simulink model "fsd_suspension"  (R2024b)
settings: Solver=ode15s  StartTime=0.0  StopTime=Tsim  FixedStep=Ts  MaxStep=1e-4  RelTol=1e-4
values from neighbouring files (symbols this model uses):
  b1 = 3500    [FSD_Analysis.m]    (also in FSD_Parameter_Sweep.m)
  b2 = 100    [FSD_Analysis.m]    (also in FSD_Parameter_Sweep.m)
  C_base = 1500    [FSD_Analysis.m]
  C_fsd = 2000    [FSD_Analysis.m]
  K_fsd = 50000    [FSD_Analysis.m]
  tau = 1/(2*pi*fc)    (= 0.0530516476973)    [FSD_Analysis.m]
undefined symbols (not defined in the file or in its folder): c_high, c_low
libraries: fl_lib x27, nesl_utility x21, sdl_lib x3
settings Model: Creator=Dinulkar  LastModifiedBy=dinul
settings DataIOCC: ReturnWorkspaceOutputs=off

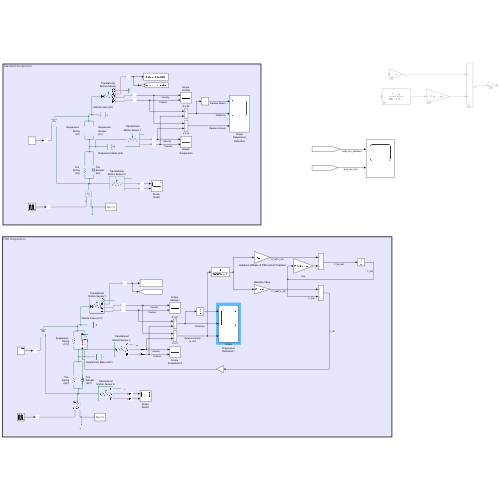
[thumbnail: Simulink's stored preview of the top-level diagram]
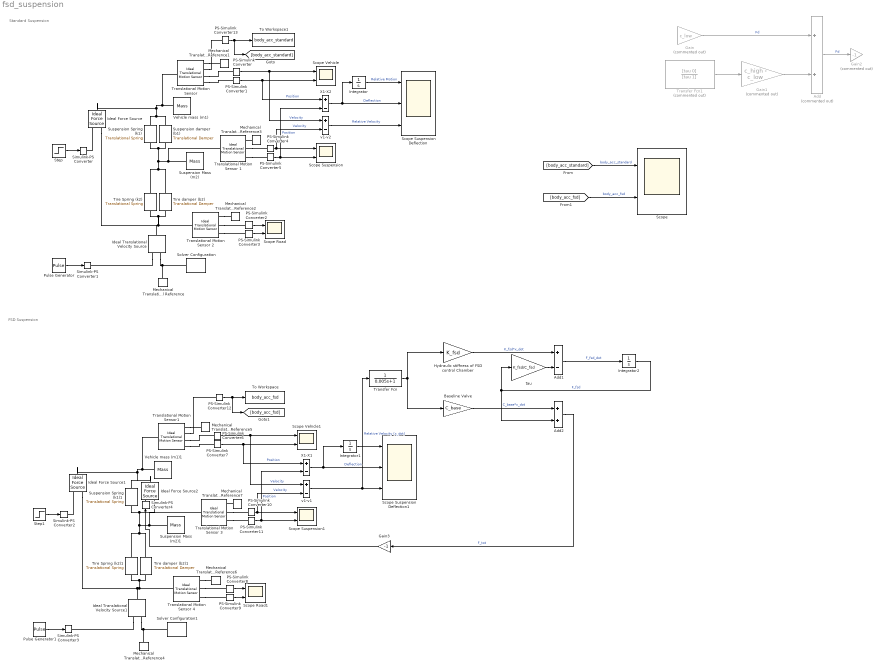
== system fsd_suspension ==
  note: FSD Suspension
  note: Standard Suspension
  Add : Sum  Commented=on
  Add1 : Sum  Inputs=+-
  Add2 : Sum
  Baseline Valve : Gain  Gain=C_base
  Gain : Gain  Commented=on  Gain=c_low
  Gain1 : Gain  Commented=on  Gain=c_high - c_low
  Gain2 : Gain  Commented=on  Gain=-1
  Gain3 : Gain  Gain=-1
  Hydraulic stiffness of FSD control Chamber : Gain  Gain=K_fsd
  Ideal Force Source : fl_lib/Mechanical/Mechanical Sources/Ideal Force Source
  Ideal Force Source1 : fl_lib/Mechanical/Mechanical Sources/Ideal Force Source
  Ideal Force Source2 : fl_lib/Mechanical/Mechanical Sources/Ideal Force Source
  Ideal Translational Velocity Source : fl_lib/Mechanical/Mechanical Sources/Ideal Translational Velocity Source
  Ideal Translational Velocity Source1 : fl_lib/Mechanical/Mechanical Sources/Ideal Translational Velocity Source
  Integrator : Integrator
  Integrator1 : Integrator
  Integrator2 : Integrator
  Mechanical Translational Reference{,1..7} (8 alike) : fl_lib/Mechanical/Translational Elements/Mechanical Translational Reference
  PS-Simulink Converter{,1..11} (12 alike) : nesl_utility/PS-Simulink Converter  PhysicalDomain=network_engine_domain  SubClassName=ps_output  LeftPortType=input  RightPortType=output  PseudoPeriodic=off  Frequencies=[]  VectorFormat=inherit  Unit=inherit  AffineConversion=off
  PS-Simulink Converter12 : nesl_utility/PS-Simulink Converter  PhysicalDomain=network_engine_domain  SubClassName=ps_output  LeftPortType=input  RightPortType=output  PseudoPeriodic=off  Frequencies=[]  VectorFormat=1-D array  Unit=inherit  AffineConversion=off
  PS-Simulink Converter13 : nesl_utility/PS-Simulink Converter  PhysicalDomain=network_engine_domain  SubClassName=ps_output  LeftPortType=input  RightPortType=output  PseudoPeriodic=off  Frequencies=[]  VectorFormat=1-D array  Unit=inherit  AffineConversion=off
  Pulse Generator : DiscretePulseGenerator  PulseType=Time based  Amplitude=0.05  PulseWidth=10  PhaseDelay=1  SampleTime=0.001
  Pulse Generator1 : DiscretePulseGenerator  PulseType=Time based  Amplitude=0.05  PulseWidth=10  PhaseDelay=1  SampleTime=0.001
  Scope : Scope  NumInputPorts=2
  Scope Suspension Deflection : Scope  NumInputPorts=3
  Scope Suspension Deflection1 : Scope  NumInputPorts=3
  Scope Road : Scope  NumInputPorts=2
  Scope Road1 : Scope  NumInputPorts=2
  Scope Suspension : Scope  NumInputPorts=2
  Scope Suspension1 : Scope  NumInputPorts=2
  Scope Vehicle : Scope  NumInputPorts=2
  Scope Vehicle1 : Scope  NumInputPorts=2
  Simulink-PS Converter : nesl_utility/Simulink-PS Converter  PhysicalDomain=network_engine_domain  SubClassName=ps_input  LeftPortType=input  RightPortType=output  PseudoPeriodic=off  Frequencies=[]  NoiseDistribution=none  NoiseParameters=[]  Unit=N  AffineConversion=on  FilteringAndDerivatives=zero  SimscapeFilterOrder=1  InputFilterTimeConstant=0.001  UdotUserProvided=0
  Simulink-PS Converter1 : nesl_utility/Simulink-PS Converter  PhysicalDomain=network_engine_domain  SubClassName=ps_input  LeftPortType=input  RightPortType=output  PseudoPeriodic=off  Frequencies=[]  NoiseDistribution=none  NoiseParameters=[]  Unit=m/s  AffineConversion=on  FilteringAndDerivatives=zero  SimscapeFilterOrder=1  InputFilterTimeConstant=0.001  UdotUserProvided=0
  Simulink-PS Converter2 : nesl_utility/Simulink-PS Converter  PhysicalDomain=network_engine_domain  SubClassName=ps_input  LeftPortType=input  RightPortType=output  PseudoPeriodic=off  Frequencies=[]  NoiseDistribution=none  NoiseParameters=[]  Unit=N  AffineConversion=on  FilteringAndDerivatives=filter  SimscapeFilterOrder=1  InputFilterTimeConstant=0.01  UdotUserProvided=0
  Simulink-PS Converter3 : nesl_utility/Simulink-PS Converter  PhysicalDomain=network_engine_domain  SubClassName=ps_input  LeftPortType=input  RightPortType=output  PseudoPeriodic=off  Frequencies=[]  NoiseDistribution=none  NoiseParameters=[]  Unit=m/s  AffineConversion=on  FilteringAndDerivatives=filter  SimscapeFilterOrder=1  InputFilterTimeConstant=0.01  UdotUserProvided=0
  Simulink-PS Converter4 : nesl_utility/Simulink-PS Converter  PhysicalDomain=network_engine_domain  SubClassName=ps_input  LeftPortType=input  RightPortType=output  PseudoPeriodic=off  Frequencies=[]  NoiseDistribution=none  NoiseParameters=[]  Unit=N  AffineConversion=off  FilteringAndDerivatives=zero  SimscapeFilterOrder=1  InputFilterTimeConstant=0.001  UdotUserProvided=0
  Solver Configuration : nesl_utility/Solver Configuration  PhysicalDomain=network_engine_domain  SubClassName=solver  LeftPortType=input  RightPortType=generic  Tones=[]  Harmonics=[]  SimulateNoise=off  Profile=off  UseLocalSampling=off  EnableSwitchedLinearOptims=on  FrequencyDomain=off  UseCCode=off  RelTol=0.001  AbsTol=0.001  MinStep=1e-09  ToWorkspace=off  RevertToSquareIcSolve=off  NumHomotopyIterations=100  PhasorMode=off  PhasorModeNumHarmonics=1  ConsistencySolver=NEWTON_XTOL_AFTER_FTOL  IndexReductionMethod=DerivativeReplacement  DoDC=off  ResidualTolerance=1e-09  ConsistencyTolSource=GLOBAL  ConsistencyAbsTol=0.001  ConsistencyRelTol=0.001  ConsistencyTolFactor=0.001  UseLocalSolver=off  LocalSolverChoice=NE_BACKWARD_EULER_ADVANCER  ResolveIndetEquations=on  FunctionEvalNumThread=1  LocalSolverSampleTime=0.001  DoFixedCost=off  MaxNonlinIter=3  MaxModeIter=2  ComputeImpulses=off  ImpulseIterations=2  LinearAlgebra=auto  LinearAlgebraNumThread=0  EquationFormulation=NE_TIME_EF  DelaysMemoryBudget=1024  AutomaticFiltering=on  FilteringTimeConstant=0.001  PartitionStorageMethod=AS_NEEDED  PartitionMemoryBudget=1024  PartitionMethod=ROBUST  MultibodyUseLocalSolver=off  MultibodyLocalSolverChoice=ODE1  MultibodyLocalSolverSampleTime=0.001
  Solver Configuration1 : nesl_utility/Solver Configuration  PhysicalDomain=network_engine_domain  SubClassName=solver  LeftPortType=input  RightPortType=generic  Tones=[]  Harmonics=[]  SimulateNoise=off  Profile=off  UseLocalSampling=off  EnableSwitchedLinearOptims=on  FrequencyDomain=off  UseCCode=off  RelTol=0.001  AbsTol=0.001  MinStep=1e-09  ToWorkspace=off  RevertToSquareIcSolve=off  NumHomotopyIterations=100  PhasorMode=off  PhasorModeNumHarmonics=1  ConsistencySolver=NEWTON_XTOL_AFTER_FTOL  IndexReductionMethod=DerivativeReplacement  DoDC=off  ResidualTolerance=1e-09  ConsistencyTolSource=GLOBAL  ConsistencyAbsTol=0.001  ConsistencyRelTol=0.001  ConsistencyTolFactor=0.001  UseLocalSolver=off  LocalSolverChoice=NE_BACKWARD_EULER_ADVANCER  ResolveIndetEquations=on  FunctionEvalNumThread=1  LocalSolverSampleTime=0.001  DoFixedCost=off  MaxNonlinIter=3  MaxModeIter=2  ComputeImpulses=off  ImpulseIterations=2  LinearAlgebra=auto  LinearAlgebraNumThread=0  EquationFormulation=NE_TIME_EF  DelaysMemoryBudget=1024  AutomaticFiltering=on  FilteringTimeConstant=0.001  PartitionStorageMethod=AS_NEEDED  PartitionMemoryBudget=1024  PartitionMethod=ROBUST  MultibodyUseLocalSolver=off  MultibodyLocalSolverChoice=ODE1  MultibodyLocalSolverSampleTime=0.001
  Step : Step  After=100  SampleTime=0
  Step1 : Step  After=100  SampleTime=0
  Suspension Spring (k1) : fl_lib/Mechanical/Translational Elements/Translational Spring  spr_rate=k1 N/m  v_specify=off  v_priority=None  v=0 m/s  v_nominal_specify=off  v_nominal_value=1  v_nominal_unit=m/s  f_specify=off  f_priority=None  f=0 N  f_nominal_specify=off  f_nominal_value=1  f_nominal_unit=N  x_specify=off  x_priority=High  x=0 m  x_nominal_specify=off  x_nominal_value=1  x_nominal_unit=m
  Suspension Spring (k1)1 : fl_lib/Mechanical/Translational Elements/Translational Spring  spr_rate=k1 N/m  v_specify=off  v_priority=None  v=0 m/s  v_nominal_specify=off  v_nominal_value=1  v_nominal_unit=m/s  f_specify=off  f_priority=None  f=0 N  f_nominal_specify=off  f_nominal_value=1  f_nominal_unit=N  x_specify=off  x_priority=High  x=0 m  x_nominal_specify=off  x_nominal_value=1  x_nominal_unit=m
  Suspension damper (b1) : sdl_lib/Couplings & Drives/Springs & Dampers/Translational Damper  D=b1 N*s/m  thermal_port=simscape.enum.thermaleffects.omit  thermal_mass=50 kJ/K  temperature_specify=off  temperature_priority=High  temperature=300 K  temperature_nominal_specify=off  temperature_nominal_value=1  temperature_nominal_unit=K
  Suspension Mass (m2) : fl_lib/Mechanical/Translational Elements/Mass  mass=m2 kg  num_ports=foundation.enum.numPorts2.one  v_specify=off  v_priority=High  v=0 m/s  v_nominal_specify=off  v_nominal_value=1  v_nominal_unit=m/s  f_specify=off  f_priority=None  f=0 N  f_nominal_specify=off  f_nominal_value=1  f_nominal_unit=N
  Suspension Mass (m2)1 : fl_lib/Mechanical/Translational Elements/Mass  mass=m2 kg  num_ports=foundation.enum.numPorts2.one  v_specify=off  v_priority=High  v=0 m/s  v_nominal_specify=off  v_nominal_value=1  v_nominal_unit=m/s  f_specify=off  f_priority=None  f=0 N  f_nominal_specify=off  f_nominal_value=1  f_nominal_unit=N
  Tire Spring (k2) : fl_lib/Mechanical/Translational Elements/Translational Spring  spr_rate=k2 N/m  v_specify=off  v_priority=None  v=0 m/s  v_nominal_specify=off  v_nominal_value=1  v_nominal_unit=m/s  f_specify=off  f_priority=None  f=0 N  f_nominal_specify=off  f_nominal_value=1  f_nominal_unit=N  x_specify=off  x_priority=High  x=0 m  x_nominal_specify=off  x_nominal_value=1  x_nominal_unit=m
  Tire Spring (k2)1 : fl_lib/Mechanical/Translational Elements/Translational Spring  spr_rate=k2 N/m  v_specify=off  v_priority=None  v=0 m/s  v_nominal_specify=off  v_nominal_value=1  v_nominal_unit=m/s  f_specify=off  f_priority=None  f=0 N  f_nominal_specify=off  f_nominal_value=1  f_nominal_unit=N  x_specify=off  x_priority=High  x=0 m  x_nominal_specify=off  x_nominal_value=1  x_nominal_unit=m
  Tire damper (b2) : sdl_lib/Couplings & Drives/Springs & Dampers/Translational Damper  D=b2 N*s/m  thermal_port=simscape.enum.thermaleffects.omit  thermal_mass=50 kJ/K  temperature_specify=off  temperature_priority=High  temperature=300 K  temperature_nominal_specify=off  temperature_nominal_value=1  temperature_nominal_unit=K
  Tire damper (b2)1 : sdl_lib/Couplings & Drives/Springs & Dampers/Translational Damper  D=b2 N*s/m  thermal_port=simscape.enum.thermaleffects.omit  thermal_mass=50 kJ/K  temperature_specify=off  temperature_priority=High  temperature=300 K  temperature_nominal_specify=off  temperature_nominal_value=1  temperature_nominal_unit=K
  To Workspace : ToWorkspace  VariableName=body_acc_fsd  SaveFormat=Structure With Time  SampleTime=-1
  To Workspace1 : ToWorkspace  VariableName=body_acc_standard  SaveFormat=Structure With Time  SampleTime=-1
  Transfer Fcn : TransferFcn  Denominator=[0.005 1]
  Transfer Fcn1 : TransferFcn  Commented=on  Numerator=[tau 0]  Denominator=[tau 1]
  Translational Motion Sensor : fl_lib/Mechanical/Mechanical Sensors/Ideal Translational Motion Sensor  reference=foundation.enum.MeasurementReference.difference  acceleration_port=true  velocity_port=true  position_port=true  offset=0 m
      settings: InternalSimscapePortConfiguration="{\"Bottom\":[],\"Left\":[{\"id\":\"R\",\"label\":\"R\",\"type\":\"foundation.mechanical.translational.translational\"}],\"Right\":[{\"id\":\"C\",\"label\":\"C\",\"type\":\"foundation.mechanical.translational.translational\"},{\"id\":\"A\",\"label\":\"A\",\"type\":\"output\"},{\"id\":\"V\",\"label\":\"V\",\"type\":\"output\"},{\"id\":\"P\",\"label\":\"P\",\"type\":\"output\"}],\"Top\":[]}"
  Translational Motion Sensor {1..4} (4 alike) : fl_lib/Mechanical/Mechanical Sensors/Ideal Translational Motion Sensor  reference=foundation.enum.MeasurementReference.difference  acceleration_port=false  velocity_port=true  position_port=true  offset=0 m
  Translational Motion Sensor1 : fl_lib/Mechanical/Mechanical Sensors/Ideal Translational Motion Sensor  reference=foundation.enum.MeasurementReference.difference  acceleration_port=true  velocity_port=true  position_port=true  offset=0 m
      settings: InternalSimscapePortConfiguration="{\"Bottom\":[],\"Left\":[{\"id\":\"R\",\"label\":\"R\",\"type\":\"foundation.mechanical.translational.translational\"}],\"Right\":[{\"id\":\"C\",\"label\":\"C\",\"type\":\"foundation.mechanical.translational.translational\"},{\"id\":\"A\",\"label\":\"A\",\"type\":\"output\"},{\"id\":\"V\",\"label\":\"V\",\"type\":\"output\"},{\"id\":\"P\",\"label\":\"P\",\"type\":\"output\"}],\"Top\":[]}"
  Vehicle mass (m1) : fl_lib/Mechanical/Translational Elements/Mass  mass=m1 kg  num_ports=foundation.enum.numPorts2.one  v_specify=off  v_priority=High  v=0 m/s  v_nominal_specify=off  v_nominal_value=1  v_nominal_unit=m/s  f_specify=off  f_priority=None  f=0 N  f_nominal_specify=off  f_nominal_value=1  f_nominal_unit=N
  Vehicle mass (m1)1 : fl_lib/Mechanical/Translational Elements/Mass  mass=m1 kg  num_ports=foundation.enum.numPorts2.one  v_specify=off  v_priority=High  v=0 m/s  v_nominal_specify=off  v_nominal_value=1  v_nominal_unit=m/s  f_specify=off  f_priority=None  f=0 N  f_nominal_specify=off  f_nominal_value=1  f_nominal_unit=N
  X1-X1 : Sum  Inputs=+-
  X1-X2 : Sum  Inputs=+-
  tau : Gain  Gain=K_fsd/C_fsd
  v1-v1 : Sum  Inputs=+-
  v1-v2 : Sum  Inputs=+-
  wires:
  Step/1 -> Simulink-PS Converter/1
  Pulse Generator/1 -> Simulink-PS Converter1/1
  PS-Simulink Converter/1 -> v1-v2/1, Scope Vehicle/1  "Velocity"
  PS-Simulink Converter1/1 -> X1-X2/1, Scope Vehicle/2  "Position"
  PS-Simulink Converter2/1 -> Scope Road/1
  PS-Simulink Converter3/1 -> Scope Road/2
  PS-Simulink Converter5/1 -> X1-X2/2, Scope Suspension/2  "Position"
  PS-Simulink Converter4/1 -> v1-v2/2, Scope Suspension/1  "Velocity"
  X1-X2/1 -> Scope Suspension Deflection/2, Integrator/1  "Deflection"
  v1-v1/1 -> Transfer Fcn/1, Scope Suspension Deflection1/3  "Relative Velocity (x_dot)"
  Integrator/1 -> Scope Suspension Deflection/1  "Relative Motion"
  Integrator1/1 -> Scope Suspension Deflection1/1
  X1-X1/1 -> Integrator1/1, Scope Suspension Deflection1/2  "Deflection"
  PS-Simulink Converter10/1 -> Scope Suspension1/1, v1-v1/2  "Velocity"
  PS-Simulink Converter11/1 -> Scope Suspension1/2, X1-X1/2  "Position"
  PS-Simulink Converter9/1 -> Scope Road1/2
  PS-Simulink Converter8/1 -> Scope Road1/1
  PS-Simulink Converter7/1 -> Scope Vehicle1/2, X1-X1/1  "Position"
  PS-Simulink Converter6/1 -> Scope Vehicle1/1, v1-v1/1  "Velocity"
  Pulse Generator1/1 -> Simulink-PS Converter3/1
  Step1/1 -> Simulink-PS Converter2/1
  PS-Simulink Converter12/1 -> [body_acc_fsd], To Workspace/1
  PS-Simulink Converter13/1 -> [body_acc_standard], To Workspace1/1
  v1-v2/1 -> Scope Suspension Deflection/3  "Relative Velocity"
  [body_acc_standard] -> Scope/1  "body_acc_standard"
  [body_acc_fsd] -> Scope/2  "body_acc_fsd"
  Hydraulic stiffness of FSD control Chamber/1 -> Add1/1  "K_fsd*x_dot"
  Add1/1 -> Integrator2/1  "F_fsd_dot"
  Integrator2/1 -> Add2/2, tau/1  "F_fsd"
  tau/1 -> Add1/2
  Add2/1 -> Gain3/1  "F_tot"
  Gain1/1 -> Add/2
  Gain/1 -> Add/1  "Fd"
  Add/1 -> Gain2/1  "Fd"
  Transfer Fcn1/1 -> Gain1/1
  Transfer Fcn/1 -> Baseline Valve/1, Hydraulic stiffness of FSD control Chamber/1
  Baseline Valve/1 -> Add2/1  "C_base*x_dot"
  Gain3/1 -> Simulink-PS Converter4/1
  connections:
  Simulink-PS Converter/RConn1 -- Ideal Force Source/RConn1
  Suspension Spring (k1)/LConn1 -- Ideal Force Source/LConn1 -- Translational Motion Sensor/LConn1 -- Vehicle mass (m1)/LConn1 -- Suspension damper (b1)/LConn1
  Suspension Spring (k1)/RConn1 -- Tire damper (b2)/LConn1 -- Tire Spring (k2)/LConn1 -- Translational Motion Sensor 1/LConn1 -- Suspension Mass (m2)/LConn1 -- Suspension damper (b1)/RConn1
  Ideal Translational Velocity Source/RConn1 -- Simulink-PS Converter1/RConn1
  Tire Spring (k2)/RConn1 -- Ideal Force Source/RConn2 -- Ideal Translational Velocity Source/LConn1 -- Translational Motion Sensor 2/LConn1 -- Tire damper (b2)/RConn1
  Mechanical Translational Reference/LConn1 -- Ideal Translational Velocity Source/RConn2 -- Solver Configuration/RConn1
  Translational Motion Sensor/RConn1 -- Mechanical Translational Reference1/LConn1
  Translational Motion Sensor 2/RConn1 -- Mechanical Translational Reference2/LConn1
  Translational Motion Sensor/RConn3 -- PS-Simulink Converter/LConn1
  Translational Motion Sensor/RConn4 -- PS-Simulink Converter1/LConn1
  Translational Motion Sensor 2/RConn2 -- PS-Simulink Converter2/LConn1
  Translational Motion Sensor 2/RConn3 -- PS-Simulink Converter3/LConn1
  Translational Motion Sensor 1/RConn3 -- PS-Simulink Converter5/LConn1
  Translational Motion Sensor 1/RConn1 -- Mechanical Translational Reference3/LConn1
  Translational Motion Sensor 1/RConn2 -- PS-Simulink Converter4/LConn1
  Ideal Force Source1/LConn1 -- Ideal Force Source2/LConn1 -- Suspension Spring (k1)1/LConn1 -- Vehicle mass (m1)1/LConn1 -- Translational Motion Sensor1/LConn1
  Suspension Spring (k1)1/RConn1 -- Ideal Force Source2/RConn2 -- Suspension Mass (m2)1/LConn1 -- Translational Motion Sensor 3/LConn1 -- Tire Spring (k2)1/LConn1 -- Tire damper (b2)1/LConn1
  Ideal Force Source1/RConn2 -- Ideal Translational Velocity Source1/LConn1 -- Translational Motion Sensor 4/LConn1 -- Tire Spring (k2)1/RConn1 -- Tire damper (b2)1/RConn1
  Ideal Translational Velocity Source1/RConn2 -- Solver Configuration1/RConn1 -- Mechanical Translational Reference4/LConn1
  Translational Motion Sensor 3/RConn2 -- PS-Simulink Converter10/LConn1
  Translational Motion Sensor 3/RConn1 -- Mechanical Translational Reference7/LConn1
  Translational Motion Sensor 4/RConn3 -- PS-Simulink Converter9/LConn1
  Translational Motion Sensor 4/RConn2 -- PS-Simulink Converter8/LConn1
  Translational Motion Sensor1/RConn4 -- PS-Simulink Converter7/LConn1
  Translational Motion Sensor1/RConn1 -- Mechanical Translational Reference5/LConn1
  Translational Motion Sensor 4/RConn1 -- Mechanical Translational Reference6/LConn1
  Translational Motion Sensor 3/RConn3 -- PS-Simulink Converter11/LConn1
  Translational Motion Sensor1/RConn3 -- PS-Simulink Converter6/LConn1
  Simulink-PS Converter2/RConn1 -- Ideal Force Source1/RConn1
  Ideal Translational Velocity Source1/RConn1 -- Simulink-PS Converter3/RConn1
  Simulink-PS Converter4/RConn1 -- Ideal Force Source2/RConn1
  Translational Motion Sensor1/RConn2 -- PS-Simulink Converter12/LConn1
  Translational Motion Sensor/RConn2 -- PS-Simulink Converter13/LConn1
